simulink model "modelo_furuta"  (R2026a)
settings: Solver=ode45  StopTime=8

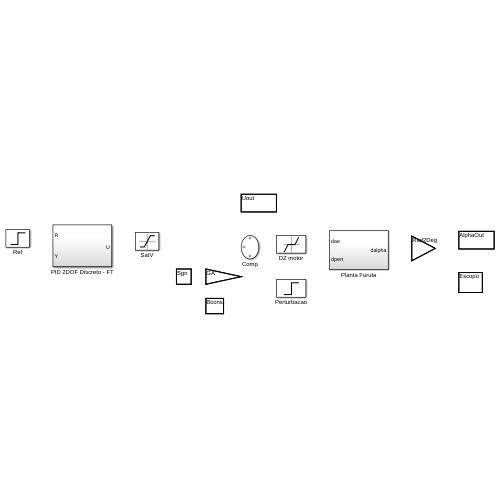
[thumbnail: Simulink's stored preview of the top-level diagram]
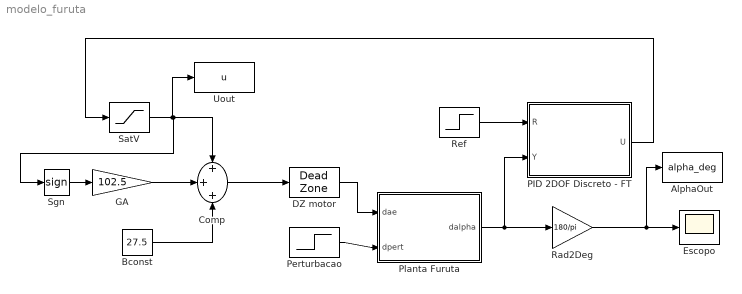
== system modelo_furuta ==
  AlphaOut : ToWorkspace  VariableName=alpha_deg  SaveFormat=Timeseries  SampleTime=-1
  Bconst : Constant  Value=27.5
  Comp : Sum  Inputs=+++
  DZ motor : DeadZone  LowerValue=-75  UpperValue=130
  Escopo : Scope
  GA : Gain  Gain=102.5
  PID 2DOF Discreto - FT : Subsystem
  Perturbacao : Step  Time=2  FinalValue=40  SampleTime=0
  Planta Furuta : Subsystem
  Rad2Deg : Gain  Gain=180/pi
  Ref : Step  Time=0  FinalValue=0  SampleTime=0
  SatV : Saturate  UpperLimit=255  LowerLimit=-255
  Sgn : Signum
  Uout : ToWorkspace  VariableName=u  SaveFormat=Timeseries  SampleTime=-1
  wires:
  Rad2Deg/1 -> Escopo/1, AlphaOut/1
  PID 2DOF Discreto - FT/1(U) -> SatV/1
  Planta Furuta/1(dalpha) -> PID 2DOF Discreto - FT/2(Y), Rad2Deg/1
  Perturbacao/1 -> Planta Furuta/2(dpert)
  Comp/1 -> DZ motor/1
  Ref/1 -> PID 2DOF Discreto - FT/1(R)
  GA/1 -> Comp/2
  SatV/1 -> Comp/1, Sgn/1, Uout/1
  DZ motor/1 -> Planta Furuta/1(dae)
  Bconst/1 -> Comp/3
  Sgn/1 -> GA/1

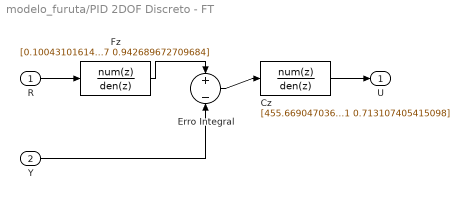
== system modelo_furuta/PID 2DOF Discreto - FT ==
  R : Inport
  Y : Inport  Port=2
  Cz : DiscreteTransferFcn  Numerator=[455.669047036076 -881.983785427658 429.554504814372]  Denominator=[1 -1.7131074054151 0.713107405415098]  SampleTime=0.02
  Erro Integral : Sum  Inputs=+-
  Fz : DiscreteTransferFcn  Numerator=[0.100431016142942 -0.147266633553737 0.0539455285269075]  Denominator=[1 -1.93557976159357 0.942689672709684]  SampleTime=0.02
  U : Outport
  wires:
  R/1 -> Fz/1
  Fz/1 -> Erro Integral/1
  Y/1 -> Erro Integral/2
  Erro Integral/1 -> Cz/1
  Cz/1 -> U/1

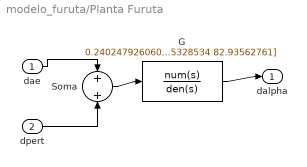
== system modelo_furuta/Planta Furuta ==
  dae : Inport
  dpert : Inport  Port=2
  G : TransferFcn  Numerator=0.240247926060648  Denominator=[1 1.35328534 82.93562761]
  Soma : Sum
  dalpha : Outport
  wires:
  dae/1 -> Soma/1
  dpert/1 -> Soma/2
  Soma/1 -> G/1
  G/1 -> dalpha/1
